simulink model "induction_motor"  (R2025b)
settings: Solver=VariableStepAuto  StartTime=0.0  StopTime=8  RelTol=1e-3
libraries: spsAsynchronousMachineSIUnitsLib x1, spsThreePhaseParallelRLCLoadLib x1, spsThreePhaseSourceLib x1, sps_lib x1
settings Model: Creator=admin  LastModifiedBy=admin
settings DataIOCC: SaveFormat=Array  ReturnWorkspaceOutputs=off

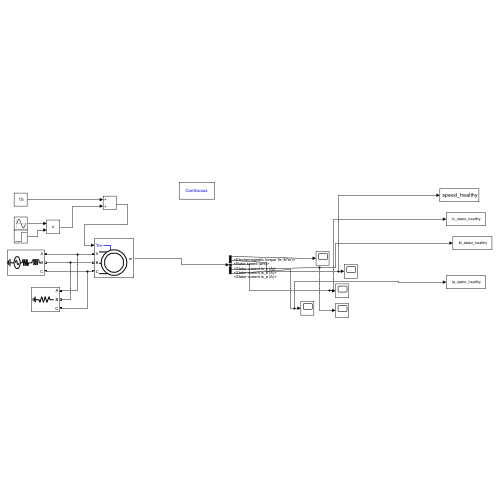
[thumbnail: Simulink's stored preview of the top-level diagram]
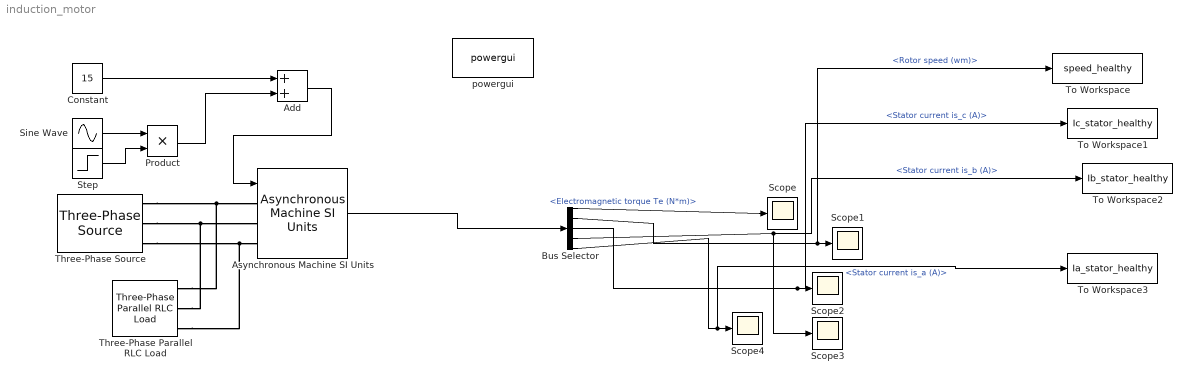
== system induction_motor ==
  Add : Sum
  Asynchronous Machine SI Units : spsAsynchronousMachineSIUnitsLib/Asynchronous Machine SI Units  RotorType=Squirrel-cage  PresetModel=No  MechanicalLoad=Torque Tm  ShowDetailedParameters=on  ReferenceFrame=Rotor  Units=SI  MeasurementBus=off  NominalParameters=[1.845e+04 400 50]  VoltageRatio=1  Stator=[0.5968 0.0003495]  Rotor=[1.2516 0.005473]  Cage1=[0.4155 0.002066]  Cage2=[0.4168 0.0003495]  Lm=0.0354  Mechanical=[0.05 0.005879 2]  PolePairs=2  InitialConditions=[0 0 0 0 0 0 0 0]  SimulateSaturation=off  Saturation=[14.03593122, 27.81365428, 53.79336849, 72.68890987, 97.98006896, 148.6815601, 215.7428561, 302.9841135, 428.7778367 ; 230, 322, 414, 460, 506, 552, 598, 644, 690]  LoadFlowParameters=1492000  TsPowergui=0  TsBlock=-1  IterativeModel=Trapezoidal non iterative  IterativeDiscreteModel=Trapezoidal non iterative  Pmec=1.492e+006
  Bus Selector : BusSelector  OutputSignals=Mechanical.Electromagnetic torque Te (N*m),Mechanical.Rotor speed (wm),Stator measurements.Stator current is_c (A),Stator measurements.Stator current is_b (A),Stator measurements.Stator current is_a (A)
  Constant : Constant  Value=15
  Product : Product
  Scope{,1..4} (5 alike) : Scope
      Scope settings: ActiveDisplayYMinimum=-1  ActiveDisplayYMaximum=1
      Scope1 settings: ActiveDisplayYMinimum=146.44865662959882  ActiveDisplayYMaximum=153.83731537236841
      Scope2 settings: ActiveDisplayYMinimum=-1  ActiveDisplayYMaximum=1  DataLoggingVariableName=ScopeData2
      Scope3 settings: ActiveDisplayYMinimum=-1  ActiveDisplayYMaximum=1  DataLoggingVariableName=ScopeData3
      Scope4 settings: ActiveDisplayYMinimum=-1  ActiveDisplayYMaximum=1  DataLoggingVariableName=ScopeData4
  Sine Wave : Sin  Amplitude=2  Frequency=1.50  SampleTime=0
  Step : Step  Time=2  SampleTime=0
  Three-Phase Parallel RLC Load : spsThreePhaseParallelRLCLoadLib/Three-Phase Parallel RLC Load  LConnTagsString=A|B|C  Configuration=Y (grounded)  NominalVoltage=400  Vabc=[1e3 1e3 1e3]  Vabcp=[1e3 1e3 1e3]  NominalFrequency=50  UnbalancedPower=off  ActivePower=1  InductivePower=0  CapacitivePower=0  Pabc=[10e3 9e3 11e3]  QLabc=[100 90 110]  QCabc=[100 90 110]  Pabcp=[10e3 9e3 11e3]  QLabcp=[100 90 110]  QCabcp=[100 90 110]  Measurements=None  LoadType=constant Z
  Three-Phase Source : spsThreePhaseSourceLib/Three-Phase Source  InternalConnection=Yg  VoltagePhases=off  Voltage=400  PhaseAngle=0  Voltage_phases=[25e3 25e3 25e3]/sqrt(3)  PhaseAngles_phases=[0 -120 +120]  Frequency=50  NonIdealSource=on  SpecifyImpedance=off  Resistance=1  Inductance=16.58e-3  ShortCircuitLevel=100e6  BaseVoltage=25e3  XRratio=7  BusType=swing  Pref=10e3  Qref=0  Prefabc=[10e3, 10e3, 10e3]  Qrefabc=[0, 0, 0]  Qmin=-inf  Qmax=inf
  To Workspace : ToWorkspace  VariableName=speed_healthy  SampleTime=-1
  To Workspace1 : ToWorkspace  VariableName=Ic_stator_healthy  SampleTime=-1
  To Workspace2 : ToWorkspace  VariableName=Ib_stator_healthy  SampleTime=-1
  To Workspace3 : ToWorkspace  VariableName=Ia_stator_healthy  SampleTime=-1
  powergui : sps_lib/powergui  Priority=1  SimulationMode=Continuous  SampleTime=50e-6  frequency=60  Iterations=50  frequencyindice=50  Pbase=100e6  ErrMax=1e-4  UnitsV=kV  UnitsW=MW  buscounter=0  FunctionMessages=off  echomessages=off  EnableUseOfTLC=off  CurrentSourceSwitches=on  DisableSnubberDevices=off  DisableRonSwitches=off  DisableVfSwitches=off  DisplayEquations=off  AutomaticDiscreteSolvers=off  SolverType=Tustin/Backward Euler (TBE)  Interpol=off  ExternalGateDelay=off  methode=off  Ts=100  x0status=blocks  SPID=on  SwTol=0  HookPort=off  NonlinearTolerance=1e-4  nMaxIteration=100  ContinueOnMaxIteration=off  RestoreLinks=warning  ResistiveCurrentMeasurement=off  Frange=[0:2:500]  Ylog=off  Xlog=on  ShowGrid=off  save=off  variable=ZData  structure=0  ZoomFFT=off  StartTime=0.0  cycles=1  DisplayStyle=1  fundamental=60  FreqAxis=off  MaxFrequency=1000  frequencyindicesteady=1  RmsSteady=1  display=off
  wires:
  Asynchronous Machine SI Units/1 -> Bus Selector/1
  Bus Selector/1 -> Scope/1  "<Electromagnetic torque Te (N*m)>"
  Bus Selector/2 -> To Workspace/1, Scope1/1  "<Rotor speed (wm)>"
  Bus Selector/3 -> To Workspace1/1, Scope2/1  "<Stator current is_c (A)>"
  Bus Selector/4 -> To Workspace2/1, Scope3/1  "<Stator current is_b (A)>"
  Bus Selector/5 -> To Workspace3/1, Scope4/1  "<Stator current is_a (A)>"
  Constant/1 -> Add/1
  Add/1 -> Asynchronous Machine SI Units/1
  Sine Wave/1 -> Product/1
  Step/1 -> Product/2
  Product/1 -> Add/2
  connections:
  Three-Phase Source/RConn1 -- Three-Phase Parallel RLC Load/LConn1 -- Asynchronous Machine SI Units/LConn1
  Three-Phase Source/RConn2 -- Three-Phase Parallel RLC Load/LConn2 -- Asynchronous Machine SI Units/LConn2
  Three-Phase Source/RConn3 -- Three-Phase Parallel RLC Load/LConn3 -- Asynchronous Machine SI Units/LConn3
